simulink model "Lab4_Digital_Control_System"  (R2023b)
settings: Solver=FixedStepAuto  StartTime=0.0  StopTime=10.0  FixedStep=0.002  RelTol=1e-3
settings Model: Creator=Liu  LastModifiedBy=Liu

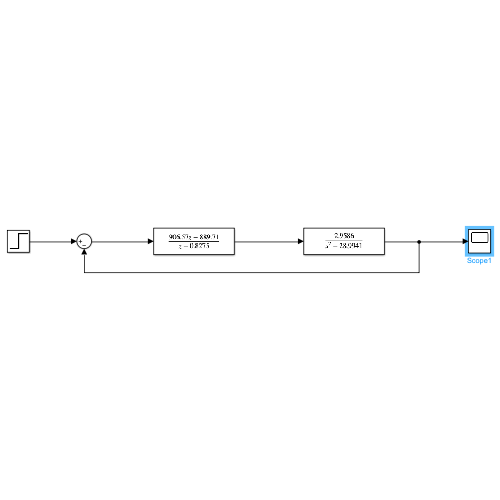
[thumbnail: Simulink's stored preview of the top-level diagram]
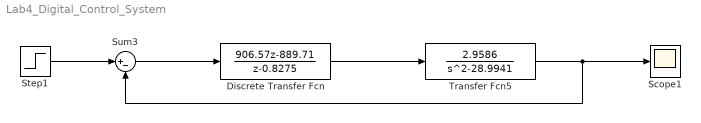
== system Lab4_Digital_Control_System ==
  Discrete Transfer Fcn : DiscreteTransferFcn  Numerator=[906.57 -889.71]  Denominator=[1 -0.8275]
  Scope1 : Scope
  Step1 : Step  SampleTime=0
  Sum3 : Sum  Inputs=|+-
  Transfer Fcn5 : TransferFcn  Numerator=[2.9586]  Denominator=[1 0 -28.9941]
  wires:
  Transfer Fcn5/1 -> Scope1/1, Sum3/2
  Step1/1 -> Sum3/1
  Sum3/1 -> Discrete Transfer Fcn/1
  Discrete Transfer Fcn/1 -> Transfer Fcn5/1
